simulink model "Bidirectional_AC_DC_full_control_V5_0_HW_Target"  (R2024a)
settings: Solver=VariableStepAuto  StartTime=0.0  StopTime=10.0  RelTol=1e-3
undefined symbols (not defined in the file): Down, GPTRIP1SEL, TZ1, Up
libraries: c2802xlib x7, c2837xDlib x7, simulink x5, slpidlib x3, spsFirstOrderFilterLib x2, spsAlphaBetaZerotodq0Lib x1
settings Model: Creator=MANSY  LastModifiedBy=MANSY

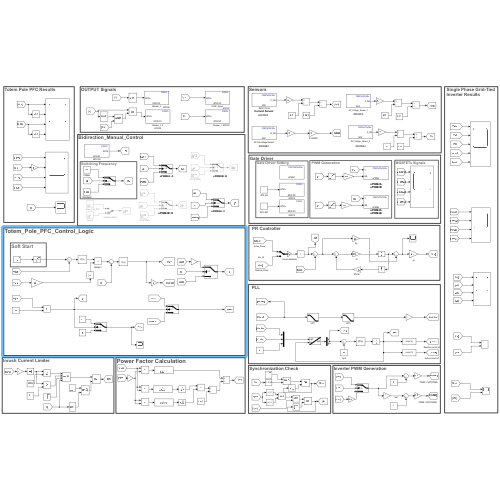
[thumbnail: Simulink's stored preview of the top-level diagram]
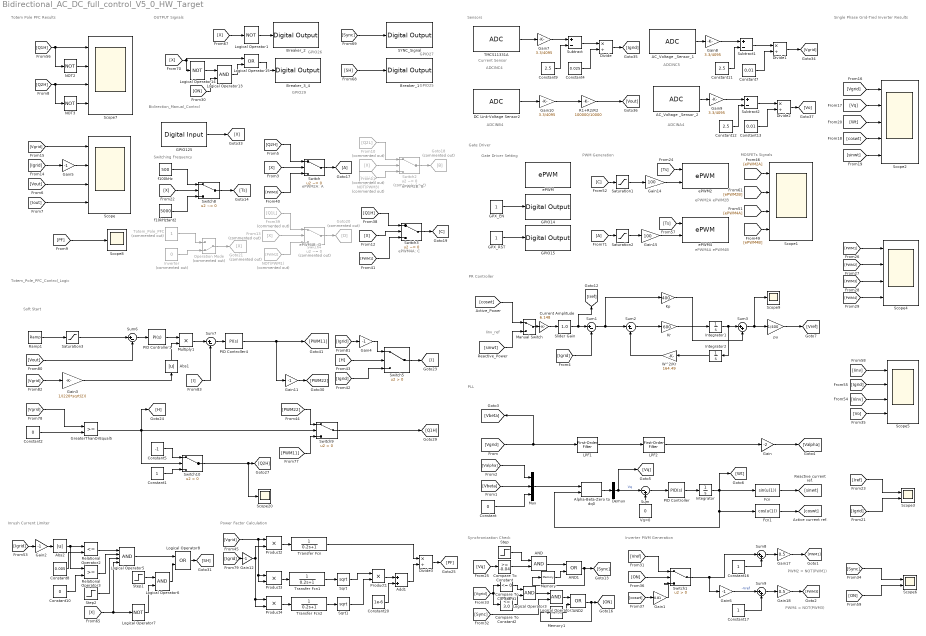
== system Bidirectional_AC_DC_full_control_V5_0_HW_Target ==
  note: Switching Frequency
  note: MOSFETs Signals
  note: OUTPUT Signals
  note: ePWM4A: C
  note: ePWM2B: B
  note: ePWM2A: A
  note: ADCINC5
  note: ADCINA4
  note: ADCINB4
  note: ADCINC4
  note: Synchronization Check
  note: PLL
  note: PR Controller
  note: Iinv_ref
  note: Bidirection_Manual_Control
  note: Inrush Current Limiter
  note: Sensors
  note: Current Sensor
  note: Gate Driver Setting
  note: ePWM2A
      | ePWM2B
  note: ePWM4A
      | ePWM4B
  note: PWM Generation
  note: Gate Driver
  note: ePWM4B: D
  note: GPIO29
  note: GPIO26
  note: GPIO27
  note: GPIO25
  note: Totem Pole PFC Results
  note: Single Phase Grid-Tied
      |  Inverter Results
  note: Soft Start
  note: Totem_Pole_PFC_Control_Logic
  note: Power Factor Calculation
  note: Inverter PWM Generation
  note: PWM2 = NOT(PWM1)
  note: PWM4 = NOT(PWM3)
  "          Totem_Pole_PFC" : Constant  Commented=on  OutDataTypeStr=boolean  SampleTime=1e-6
  AC_Voltage _Sensor_1 : c2802xlib/ADC  blkParamProc=C2000_Type4  ADCModule=C  samplingMode=Single sample mode  ADCResolution=12-bit (Single-ended input)  useSOC1=SOC1  useSOC2=SOC0_SOC1  SOCAcquisitionWindow=15  SOCTriggerSource=Software  SOCInterruptTrigger=No ADCINT  Ts=0.001  dType=uint16  postInterrupt=off  interruptSel=ADCINT1  ADCINTContinuous=on  endma=off  chdma=1  conv1=ADCINA0  conv2=ADCINA0 and ADCINB0  conv1_Type4=ADCIN5  conv2_Type4=ADCIN0 and ADCIN1
      settings: LibrarySourceBlock=c2837xDlib/ADC
  AC_Voltage _Sensor_2 : c2802xlib/ADC  blkParamProc=C2000_Type4  ADCModule=A  samplingMode=Single sample mode  ADCResolution=12-bit (Single-ended input)  useSOC1=SOC0  useSOC2=SOC0_SOC1  SOCAcquisitionWindow=15  SOCTriggerSource=Software  SOCInterruptTrigger=No ADCINT  Ts=0.001  dType=uint16  postInterrupt=off  interruptSel=ADCINT1  ADCINTContinuous=on  endma=off  chdma=1  conv1=ADCINA0  conv2=ADCINA0 and ADCINB0  conv1_Type4=ADCIN4  conv2_Type4=ADCIN0 and ADCIN1
      settings: LibrarySourceBlock=c2837xDlib/ADC
  AND : Logic  AllPortsSameDT=off  OutDataTypeStr=boolean
  AND1 : Logic  Operator=OR  AllPortsSameDT=off  OutDataTypeStr=boolean
  AND2 : Logic  Operator=OR  AllPortsSameDT=off  OutDataTypeStr=boolean
  Abs1 : Abs  SaturateOnIntegerOverflow=off
  Abs2 : Abs  SaturateOnIntegerOverflow=off
  Add1 : Sum
  Alpha-Beta-Zero to dq0 : spsAlphaBetaZerotodq0Lib/Alpha-Beta-Zero to dq0  Alignment=90 degrees behind phase A axis
  Breaker_1 : c2837xDlib/Digital Output  GPIO_Number=GPIO24~GPIO31  GPIO_Bit0=off  GPIO_BIT0_Toggle=off  GPIO_Bit1=on  GPIO_BIT1_Toggle=off  GPIO_Bit2=off  GPIO_BIT2_Toggle=off  GPIO_Bit3=off  GPIO_BIT3_Toggle=off  GPIO_Bit4=off  GPIO_BIT4_Toggle=off  GPIO_Bit5=off  GPIO_BIT5_Toggle=off  GPIO_Bit6=off  GPIO_BIT6_Toggle=off  GPIO_Bit7=off  GPIO_BIT7_Toggle=off
  Breaker_2 : c2837xDlib/Digital Output  GPIO_Number=GPIO24~GPIO31  GPIO_Bit0=off  GPIO_BIT0_Toggle=off  GPIO_Bit1=off  GPIO_BIT1_Toggle=off  GPIO_Bit2=on  GPIO_BIT2_Toggle=off  GPIO_Bit3=off  GPIO_BIT3_Toggle=off  GPIO_Bit4=off  GPIO_BIT4_Toggle=off  GPIO_Bit5=off  GPIO_BIT5_Toggle=off  GPIO_Bit6=off  GPIO_BIT6_Toggle=off  GPIO_Bit7=off  GPIO_BIT7_Toggle=off
  Breaker_3_4 : c2837xDlib/Digital Output  GPIO_Number=GPIO24~GPIO31  GPIO_Bit0=off  GPIO_BIT0_Toggle=off  GPIO_Bit1=off  GPIO_BIT1_Toggle=off  GPIO_Bit2=off  GPIO_BIT2_Toggle=off  GPIO_Bit3=off  GPIO_BIT3_Toggle=off  GPIO_Bit4=off  GPIO_BIT4_Toggle=off  GPIO_Bit5=on  GPIO_BIT5_Toggle=off  GPIO_Bit6=off  GPIO_BIT6_Toggle=off  GPIO_Bit7=off  GPIO_BIT7_Toggle=off
  Compare To Constant : simulink/Logic and Bit Operations/Compare To Constant  relop=>=  const=-0.04  OutDataTypeStr=boolean
  Compare To Constant1 : simulink/Logic and Bit Operations/Compare To Constant  relop=<=  const=0  OutDataTypeStr=boolean
  Compare To Constant2 : simulink/Logic and Bit Operations/Compare To Constant  relop=<=  const=3.0  OutDataTypeStr=boolean
  Constant : Constant  Value=0
  Constant1 : Constant
  Constant10 : Constant  Value=0
  Constant11 : Constant  Value=2.5
  Constant12 : Constant  Value=2.5
  Constant13 : Constant  Value=0.01
  Constant16 : Constant
  Constant17 : Constant
  Constant2 : Constant  Value=0
  Constant20 : Constant  Value=1e-6
  Constant4 : Constant  Value=0.025
  Constant5 : Constant  Value=-1
  Constant7 : Constant  Value=0.01
  Constant8 : Constant  Value=0.005
  Constant9 : Constant  Value=2.5
  Current Amplitude : Gain  Gain=6.148
  DC Link-Voltage Sensor2 : c2802xlib/ADC  blkParamProc=C2000_Type4  ADCModule=B  samplingMode=Single sample mode  ADCResolution=12-bit (Single-ended input)  useSOC1=SOC1  useSOC2=SOC0_SOC1  SOCAcquisitionWindow=15  SOCTriggerSource=Software  SOCInterruptTrigger=No ADCINT  Ts=0.001  dType=uint16  postInterrupt=off  interruptSel=ADCINT1  ADCINTContinuous=on  endma=off  chdma=1  conv1=ADCINA0  conv2=ADCINA0 and ADCINB0  conv1_Type4=ADCIN4  conv2_Type4=ADCIN0 and ADCIN1
      settings: LibrarySourceBlock=c2837xDlib/ADC
  Demux : Demux  Outputs=3
  Divide{,1..3} (4 alike) : Product  Inputs=*/
  Fcn : Fcn  Expr=sin(u(1))
  Fcn1 : Fcn  Expr=cos(u(1))
  From10 : From  Commented=on  GotoTag=Q2L
  From11 : From  Commented=on  GotoTag=X
  From13 : From  Commented=on  GotoTag=X
  From39 : From  Commented=on  GotoTag=Q1L
  From71 : From
  GPIO125 : c2837xDlib/Digital Input  GPIO_Number=GPIO120~GPIO127  GPIO_Bit0=off  GPIO_Bit1=off  GPIO_Bit2=off  GPIO_Bit3=off  GPIO_Bit4=off  GPIO_Bit5=on  GPIO_Bit6=off  GPIO_Bit7=off  sampleTime=0.1  dataType=auto  GPIO_Bit0_Qualification=Sync to SYSCLKOUT  GPIO_Bit1_Qualification=Sync to SYSCLKOUT  GPIO_Bit2_Qualification=Sync to SYSCLKOUT  GPIO_Bit3_Qualification=Sync to SYSCLKOUT  GPIO_Bit4_Qualification=Sync to SYSCLKOUT  GPIO_Bit5_Qualification=Sync to SYSCLKOUT  GPIO_Bit6_Qualification=Sync to SYSCLKOUT  GPIO_Bit7_Qualification=Sync to SYSCLKOUT  Qualification_Period=-1
  GPIO14 : c2837xDlib/Digital Output  GPIO_Number=GPIO8~GPIO15  GPIO_Bit0=off  GPIO_BIT0_Toggle=off  GPIO_Bit1=off  GPIO_BIT1_Toggle=off  GPIO_Bit2=off  GPIO_BIT2_Toggle=off  GPIO_Bit3=off  GPIO_BIT3_Toggle=off  GPIO_Bit4=off  GPIO_BIT4_Toggle=off  GPIO_Bit5=off  GPIO_BIT5_Toggle=off  GPIO_Bit6=on  GPIO_BIT6_Toggle=off  GPIO_Bit7=off  GPIO_BIT7_Toggle=off
  GPIO15 : c2837xDlib/Digital Output  GPIO_Number=GPIO8~GPIO15  GPIO_Bit0=off  GPIO_BIT0_Toggle=off  GPIO_Bit1=off  GPIO_BIT1_Toggle=off  GPIO_Bit2=off  GPIO_BIT2_Toggle=off  GPIO_Bit3=off  GPIO_BIT3_Toggle=off  GPIO_Bit4=off  GPIO_BIT4_Toggle=off  GPIO_Bit5=off  GPIO_BIT5_Toggle=off  GPIO_Bit6=off  GPIO_BIT6_Toggle=off  GPIO_Bit7=on  GPIO_BIT7_Toggle=off
  GPX_EN : Constant  SampleTime=1e-5
  GPX_RST : Constant  SampleTime=1e-5
  Gain : Gain  Gain=-2
  Gain1 : Gain  Gain=0.81
  Gain{7..10} (4 alike) : Gain  Gain=3.3/4095
  Gain{2,4..6,11..12} (6 alike) : Gain  Gain=-1
  Gain14 : Gain  Gain=100
  Gain15 : Gain  Gain=100
  Gain17 : Gain  Gain=0.5
  Gain18 : Gain  Gain=0.5
  Gain3 : Gain  Gain=1/(220*sqrt(2))
  Goto17 : Goto
  Goto18 : Goto  Commented=on  GotoTag=B
  Goto20 : Goto  Commented=on  GotoTag=D
  Goto21 : Goto  Commented=on  GotoTag=X
  GreaterThanOrEqual5 : RelationalOperator  OutDataTypeStr=boolean  RndMeth=Simplest  InputSameDT=off
  Integrator : Integrator
  Integrator1 : Integrator
  Integrator2 : Integrator
  Inverter : Constant  Commented=on  Value=0  OutDataTypeStr=boolean  SampleTime=1e-6
  Kp : Gain  Gain=400
  Kr : Gain  Gain=600
  LPF1 : spsFirstOrderFilterLib/First-Order Filter  FilterType=Lowpass  Tc=1/(2*pi*50)  Ts=0  Initialize=off  Vac_Init=[0, 0, 60]  Vdc_Init=0  PlotResponse=off  FreqRange="[0,  200,  1]"
  LPF2 : spsFirstOrderFilterLib/First-Order Filter  FilterType=Lowpass  Tc=1/(2*pi*50)  Ts=0  Initialize=off  Vac_Init=[0, 0, 60]  Vdc_Init=0  PlotResponse=off  FreqRange="[0,  200,  1]"
  Logical Operator1 : Logic  Operator=NOT  AllPortsSameDT=off  OutDataTypeStr=boolean
  Logical Operator{2..3,6,13} (4 alike) : Logic  AllPortsSameDT=off  OutDataTypeStr=boolean
  Logical Operator14 : Logic  Operator=NOT  AllPortsSameDT=off  OutDataTypeStr=boolean
  Logical Operator15 : Logic  Operator=OR  AllPortsSameDT=off  OutDataTypeStr=boolean
  Logical Operator5 : Logic  Inputs=4  AllPortsSameDT=off  OutDataTypeStr=boolean
  Logical Operator7 : Logic  Operator=NOT  AllPortsSameDT=off  OutDataTypeStr=boolean
  Logical Operator8 : Logic  Operator=OR  AllPortsSameDT=off  OutDataTypeStr=boolean
  Manual Switch : ManualSwitch
  Memory : Memory
  Memory1 : Memory
  Multiply1 : Product
  Mux : Mux  Inputs=3
  NOT(PWM1) : From  Commented=on  GotoTag=PWM2
  NOT(PWM3) : From  Commented=on  GotoTag=PWM4
  NOT2 : Logic  Operator=NOT  AllPortsSameDT=off  OutDataTypeStr=boolean
  NOT3 : Logic  Operator=NOT  AllPortsSameDT=off  OutDataTypeStr=boolean
  Operation Mode : ManualSwitch  Commented=on  CurrentSetting=0
  PID Controller : slpidlib/PID Controller  Controller=PID  Form=Parallel  TimeDomain=Continuous-time  UseExternalTs=off  SampleTime=-1  IntegratorMethod=Forward Euler  FilterMethod=Forward Euler  ControllerParametersSource=internal  P=100  I=10000  UseKiTs=off  D=0  UseExternalDerivativeSource=off  N=100  UseFilter=on  TunerSelectOption=Transfer Function Based (PID Tuner App)  InitialConditionSource=internal  InitialConditionForIntegrator=0  InitialConditionForFilter=0  DifferentiatorICPrevScaledInput=0  ExternalReset=none  TrackingMode=off  Kt=1  LimitOutput=off  SatLimitsSource=internal  UpperSaturationLimit=inf  LowerSaturationLimit=-inf  LinearizeAsGain=on  AntiWindupMode=none  Kb=1  LimitIntegrator=off  UpperIntegratorSaturationLimit=inf  LowerIntegratorSaturationLimit=-inf  POutMin=[]  POutMax=[]  IOutMin=[]  IOutMax=[]  DOutMin=[]  DOutMax=[]  NOutMin=[]  NOutMax=[]  SumOutMin=[]  SumOutMax=[]  SaturationOutMin=[]  SaturationOutMax=[]  PParamMin=[]  PParamMax=[]  IParamMin=[]  IParamMax=[]  DParamMin=[]  DParamMax=[]  NParamMin=[]  NParamMax=[]  KbParamMin=[]  KbParamMax=[]  KtParamMin=[]  KtParamMax=[]  KbOutMin=[]  KbOutMax=[]  KtOutMin=[]  KtOutMax=[]  IntegratorOutMin=[]  IntegratorOutMax=[]  FilterOutMin=[]  FilterOutMax=[]  SumI1OutMin=[]  SumI1OutMax=[]  SumI2OutMin=[]  SumI2OutMax=[]  SumI3OutMin=[]  SumI3OutMax=[]  SumI4OutMin=[]  SumI4OutMax=[]  SumDOutMin=[]  SumDOutMax=[]  DifferentiatorOutMin=[]  DifferentiatorOutMax=[]  FilterDiffOutCoefMin=[]  FilterDiffOutCoefMax=[]  ReciprocalOutMin=[]  ReciprocalOutMax=[]  SumDenOutMin=[]  SumDenOutMax=[]  SumNumOutMin=[]  SumNumOutMax=[]  DivideOutMin=[]  DivideOutMax=[]  UdiffTsProdOutMin=[]  UdiffTsProdOutMax=[]  NTsProdOutMin=[]  NTsProdOutMax=[]  UintegralTsProdOutMin=[]  UintegralTsProdOutMax=[]  UngainTsProdOutMin=[]  UngainTsProdOutMax=[]  ClampingZeroOutDataTypeStr=Inherit: Inherit via back propagation  ClampingZeroOutMin=[]  ClampingZeroOutMax=[]  FilterDenConstantOutDataTypeStr=Inherit: Inherit via back propagation  FilterDenConstantOutMin=[]  FilterDenConstantOutMax=[]  PCopyOutDataTypeStr=Inherit: Inherit via back propagation  PCopyOutMin=[]  PCopyOutMax=[]  NCopyOutDataTypeStr=Inherit: Inherit via back propagation  NCopyOutMin=[]  NCopyOutMax=[]  IntegratorContinuousStateAttributes=''  IntegratorStateMustResolveToSignalObject=off  IntegratorRTWStateStorageClass=Auto  FilterContinuousStateAttributes=''  FilterStateMustResolveToSignalObject=off  FilterRTWStateStorageClass=Auto  ParallelPVariant=InternalParameters  IdealPVariant=Disabled  IVariant=InternalParameters  DVariant=InternalParameters  IntegratorVariant=Continuous  SatVariant=Disabled  AWVariant=Passthrough  PCopyVariant=Disabled  TRVariant=Disabled  FdbkBlocksVariant=Forward  IdealPFdbkVariant=Disabled  SatFdbkVariant=Disabled  DerivativeFilterVariant=ContFilter  NVariant=InternalParameters  NCopyVariant=Disabled  FilterICVariant=InternalICsFilter  IntegratorICVariant=InternalICs  ExternalResetVariant=Disabled  TRSumVariant=Passthrough  SumFdbkVariant=Disabled  SumVariant=Sum_PID  TsampFilterVariant=InternalTs  TsampNgainVariant=Passthrough  TsampIntegralVariant=Disabled_SignalSpec  ExternalSaturationOutDataTypeStr=Inherit: Same as second input  DerivativeSourceVariant=ErrorSignal
  PID Controller1 : slpidlib/PID Controller  Controller=PI  Form=Parallel  TimeDomain=Continuous-time  UseExternalTs=off  SampleTime=-1  IntegratorMethod=Forward Euler  FilterMethod=Forward Euler  ControllerParametersSource=internal  P=.1  I=0.75  UseKiTs=off  D=0  UseExternalDerivativeSource=off  N=100  UseFilter=on  TunerSelectOption=Transfer Function Based (PID Tuner App)  InitialConditionSource=internal  InitialConditionForIntegrator=0  InitialConditionForFilter=0  DifferentiatorICPrevScaledInput=0  ExternalReset=none  TrackingMode=off  Kt=1  LimitOutput=off  SatLimitsSource=internal  UpperSaturationLimit=inf  LowerSaturationLimit=-inf  LinearizeAsGain=on  AntiWindupMode=none  Kb=1  LimitIntegrator=off  UpperIntegratorSaturationLimit=inf  LowerIntegratorSaturationLimit=-inf  POutMin=[]  POutMax=[]  IOutMin=[]  IOutMax=[]  DOutMin=[]  DOutMax=[]  NOutMin=[]  NOutMax=[]  SumOutMin=[]  SumOutMax=[]  SaturationOutMin=[]  SaturationOutMax=[]  PParamMin=[]  PParamMax=[]  IParamMin=[]  IParamMax=[]  DParamMin=[]  DParamMax=[]  NParamMin=[]  NParamMax=[]  KbParamMin=[]  KbParamMax=[]  KtParamMin=[]  KtParamMax=[]  KbOutMin=[]  KbOutMax=[]  KtOutMin=[]  KtOutMax=[]  IntegratorOutMin=[]  IntegratorOutMax=[]  FilterOutMin=[]  FilterOutMax=[]  SumI1OutMin=[]  SumI1OutMax=[]  SumI2OutMin=[]  SumI2OutMax=[]  SumI3OutMin=[]  SumI3OutMax=[]  SumI4OutMin=[]  SumI4OutMax=[]  SumDOutMin=[]  SumDOutMax=[]  DifferentiatorOutMin=[]  DifferentiatorOutMax=[]  FilterDiffOutCoefMin=[]  FilterDiffOutCoefMax=[]  ReciprocalOutMin=[]  ReciprocalOutMax=[]  SumDenOutMin=[]  SumDenOutMax=[]  SumNumOutMin=[]  SumNumOutMax=[]  DivideOutMin=[]  DivideOutMax=[]  UdiffTsProdOutMin=[]  UdiffTsProdOutMax=[]  NTsProdOutMin=[]  NTsProdOutMax=[]  UintegralTsProdOutMin=[]  UintegralTsProdOutMax=[]  UngainTsProdOutMin=[]  UngainTsProdOutMax=[]  ClampingZeroOutDataTypeStr=Inherit: Inherit via back propagation  ClampingZeroOutMin=[]  ClampingZeroOutMax=[]  FilterDenConstantOutDataTypeStr=Inherit: Inherit via back propagation  FilterDenConstantOutMin=[]  FilterDenConstantOutMax=[]  PCopyOutDataTypeStr=Inherit: Inherit via back propagation  PCopyOutMin=[]  PCopyOutMax=[]  NCopyOutDataTypeStr=Inherit: Inherit via back propagation  NCopyOutMin=[]  NCopyOutMax=[]  IntegratorContinuousStateAttributes=''  IntegratorStateMustResolveToSignalObject=off  IntegratorRTWStateStorageClass=Auto  FilterContinuousStateAttributes=''  FilterStateMustResolveToSignalObject=off  FilterRTWStateStorageClass=Auto  ParallelPVariant=InternalParameters  IdealPVariant=Disabled  IVariant=InternalParameters  DVariant=Disabled  IntegratorVariant=Continuous  SatVariant=Disabled  AWVariant=Passthrough  PCopyVariant=Disabled  TRVariant=Disabled  FdbkBlocksVariant=Forward  IdealPFdbkVariant=Disabled  SatFdbkVariant=Disabled  DerivativeFilterVariant=Disabled  NVariant=Disabled  NCopyVariant=Disabled_SignalSpec  FilterICVariant=Disabled  IntegratorICVariant=InternalICs  ExternalResetVariant=Disabled  TRSumVariant=Passthrough  SumFdbkVariant=Disabled  SumVariant=Sum_PI  TsampFilterVariant=InternalTs  TsampNgainVariant=Passthrough  TsampIntegralVariant=Disabled_SignalSpec  ExternalSaturationOutDataTypeStr=Inherit: Same as second input  DerivativeSourceVariant=Disabled
  PID Controller4 : slpidlib/PID Controller  Controller=PI  Form=Parallel  TimeDomain=Continuous-time  UseExternalTs=off  SampleTime=-1  IntegratorMethod=Forward Euler  FilterMethod=Forward Euler  ControllerParametersSource=internal  P=600  I=100  UseKiTs=off  D=0  UseExternalDerivativeSource=off  N=100  UseFilter=on  TunerSelectOption=Transfer Function Based (PID Tuner App)  InitialConditionSource=internal  InitialConditionForIntegrator=0  InitialConditionForFilter=0  DifferentiatorICPrevScaledInput=0  ExternalReset=none  TrackingMode=off  Kt=1  LimitOutput=off  SatLimitsSource=internal  UpperSaturationLimit=.99  LowerSaturationLimit=0  LinearizeAsGain=on  AntiWindupMode=none  Kb=1  LimitIntegrator=off  UpperIntegratorSaturationLimit=inf  LowerIntegratorSaturationLimit=-inf  POutMin=[]  POutMax=[]  IOutMin=[]  IOutMax=[]  DOutMin=[]  DOutMax=[]  NOutMin=[]  NOutMax=[]  SumOutMin=[]  SumOutMax=[]  SaturationOutMin=[]  SaturationOutMax=[]  PParamMin=[]  PParamMax=[]  IParamMin=[]  IParamMax=[]  DParamMin=[]  DParamMax=[]  NParamMin=[]  NParamMax=[]  KbParamMin=[]  KbParamMax=[]  KtParamMin=[]  KtParamMax=[]  KbOutMin=[]  KbOutMax=[]  KtOutMin=[]  KtOutMax=[]  IntegratorOutMin=[]  IntegratorOutMax=[]  FilterOutMin=[]  FilterOutMax=[]  SumI1OutMin=[]  SumI1OutMax=[]  SumI2OutMin=[]  SumI2OutMax=[]  SumI3OutMin=[]  SumI3OutMax=[]  SumI4OutMin=[]  SumI4OutMax=[]  SumDOutMin=[]  SumDOutMax=[]  DifferentiatorOutMin=[]  DifferentiatorOutMax=[]  FilterDiffOutCoefMin=[]  FilterDiffOutCoefMax=[]  ReciprocalOutMin=[]  ReciprocalOutMax=[]  SumDenOutMin=[]  SumDenOutMax=[]  SumNumOutMin=[]  SumNumOutMax=[]  DivideOutMin=[]  DivideOutMax=[]  UdiffTsProdOutMin=[]  UdiffTsProdOutMax=[]  NTsProdOutMin=[]  NTsProdOutMax=[]  UintegralTsProdOutMin=[]  UintegralTsProdOutMax=[]  UngainTsProdOutMin=[]  UngainTsProdOutMax=[]  ClampingZeroOutDataTypeStr=Inherit: Inherit via back propagation  ClampingZeroOutMin=[]  ClampingZeroOutMax=[]  FilterDenConstantOutDataTypeStr=Inherit: Inherit via back propagation  FilterDenConstantOutMin=[]  FilterDenConstantOutMax=[]  PCopyOutDataTypeStr=Inherit: Inherit via back propagation  PCopyOutMin=[]  PCopyOutMax=[]  NCopyOutDataTypeStr=Inherit: Inherit via back propagation  NCopyOutMin=[]  NCopyOutMax=[]  IntegratorContinuousStateAttributes=''  IntegratorStateMustResolveToSignalObject=off  IntegratorRTWStateStorageClass=Auto  FilterContinuousStateAttributes=''  FilterStateMustResolveToSignalObject=off  FilterRTWStateStorageClass=Auto  ParallelPVariant=InternalParameters  IdealPVariant=Disabled  IVariant=InternalParameters  DVariant=Disabled  IntegratorVariant=Continuous  SatVariant=Disabled  AWVariant=Passthrough  PCopyVariant=Disabled  TRVariant=Disabled  FdbkBlocksVariant=Forward  IdealPFdbkVariant=Disabled  SatFdbkVariant=Disabled  DerivativeFilterVariant=Disabled  NVariant=Disabled  NCopyVariant=Disabled_SignalSpec  FilterICVariant=Disabled  IntegratorICVariant=InternalICs  ExternalResetVariant=Disabled  TRSumVariant=Passthrough  SumFdbkVariant=Disabled  SumVariant=Sum_PI  TsampFilterVariant=InternalTs  TsampNgainVariant=Passthrough  TsampIntegralVariant=Disabled_SignalSpec  ExternalSaturationOutDataTypeStr=Inherit: Same as second input  DerivativeSourceVariant=Disabled
  Product{1..4} (4 alike) : Product
  R1+R2/R2 : Gain  Gain=100000/10000
  Ramp1 : simulink/Sources/Ramp  slope=4000  start=0  InitialOutput=0
  Relational Operator2 : RelationalOperator  Operator=<=  OutDataTypeStr=boolean  RndMeth=Simplest  InputSameDT=off
  Relational Operator3 : RelationalOperator  OutDataTypeStr=boolean  RndMeth=Simplest  InputSameDT=off
  "SYNC_Signal  " : c2837xDlib/Digital Output  GPIO_Number=GPIO24~GPIO31  GPIO_Bit0=off  GPIO_BIT0_Toggle=off  GPIO_Bit1=off  GPIO_BIT1_Toggle=off  GPIO_Bit2=off  GPIO_BIT2_Toggle=off  GPIO_Bit3=on  GPIO_BIT3_Toggle=off  GPIO_Bit4=off  GPIO_BIT4_Toggle=off  GPIO_Bit5=off  GPIO_BIT5_Toggle=off  GPIO_Bit6=off  GPIO_BIT6_Toggle=off  GPIO_Bit7=off  GPIO_BIT7_Toggle=off
  Saturation1 : Saturate  UpperLimit=1  LowerLimit=0
  Saturation2 : Saturate  UpperLimit=1  LowerLimit=0
  Saturation3 : Saturate  UpperLimit=400  LowerLimit=0
  Scope{,1,4..5,7} (5 alike) : Scope  NumInputPorts=4
  Scope2 : Scope  NumInputPorts=5
  Scope20 : Scope
  Scope3 : Scope  NumInputPorts=2
  Scope6 : Scope  NumInputPorts=2
  Scope8 : Scope
  Scope9 : Scope
  Slider Gain : simulink/Math Operations/Slider Gain  gain=1.0  low=0  high=1
  Sqrt : Sqrt
  Sqrt1 : Sqrt
  Step : Step  Time=0.02  SampleTime=0
  Step1 : Step  Time=0.005  SampleTime=0
  Step2 : Step  Time=0.14  SampleTime=0
  Subtract : Sum  Inputs=+-
  Subtract1 : Sum  Inputs=+-
  Subtract2 : Sum  Inputs=+-
  Sum : Sum  Inputs=|-+
  Sum{1..2,6..7} (4 alike) : Sum  Inputs=|+-
  Sum3 : Sum  Inputs=|++
  Sum8 : Sum  Inputs=|++
  Sum9 : Sum  Inputs=|++
  Switch : Switch  Criteria=u2 ~= 0  SaturateOnIntegerOverflow=off  InputSameDT=off
  Switch{1,5,9..10} (4 alike) : Switch  Criteria=u2 > Threshold  SaturateOnIntegerOverflow=off  InputSameDT=off
  Switch2 : Switch  Commented=on  Criteria=u2 ~= 0  SaturateOnIntegerOverflow=off  InputSameDT=off
  Switch3 : Switch  Criteria=u2 ~= 0  SaturateOnIntegerOverflow=off  InputSameDT=off
  Switch4 : Switch  Commented=on  Criteria=u2 ~= 0  SaturateOnIntegerOverflow=off  InputSameDT=off
  Switch8 : Switch  Criteria=u2 ~= 0  SaturateOnIntegerOverflow=off  InputSameDT=off
  TMCS11331A : c2802xlib/ADC  blkParamProc=C2000_Type4  ADCModule=C  samplingMode=Single sample mode  ADCResolution=12-bit (Single-ended input)  useSOC1=SOC0  useSOC2=SOC0_SOC1  SOCAcquisitionWindow=15  SOCTriggerSource=Software  SOCInterruptTrigger=No ADCINT  Ts=0.001  dType=uint16  postInterrupt=off  interruptSel=ADCINT1  ADCINTContinuous=on  endma=off  chdma=1  conv1=ADCINA0  conv2=ADCINA0 and ADCINB0  conv1_Type4=ADCIN4  conv2_Type4=ADCIN0 and ADCIN1
      settings: LibrarySourceBlock=c2837xDlib/ADC
  Transfer Fcn : TransferFcn  Denominator=[0.2 1]
  Transfer Fcn1 : TransferFcn  Denominator=[0.2 1]
  Transfer Fcn2 : TransferFcn  Denominator=[0.2 1]
  Vq=0 : Constant  Value=0
  W^2/Kr : Gain  Gain=164.49
  ePWM : c2802xlib/ePWM  PwmType=C2000_Type4  useModule=ePWM1  ePWMxLINKTBPRD=Not Linked  periodUnits=Clock cycles  timerSource=Specify via dialog  timerPeriod_clk=100  timerPeriod_sec=0.0001  tbshadow=Counter equals to zero  countingMode=Up-Down  phaseActiveEnable=Disable  phaseDirection=Count down after sync  phaseActive=0  synchronizationEnable=off  dcaevt1Sync=off  dcbevt1Sync=off  synchronizationOption=Disable  dcbevt1SyncOut=off  dcaevt1SyncOut=off  cmpdSyncOut=off  cmpcSyncOut=off  cmpbSyncOut=off  zeroSyncOut=off  swfSyncOut=off  perSynchronizationOption=Counter equals to period (CTR=PRD)  clockPrescale=1  HSclockPrescale=1  enswap=off  ePWMxAStatus=on  ePWMxAactionLogic1=Do nothing  ePWMxAactionLogic2=Do nothing  ePWMxAactionLogic3=Clear  ePWMxAactionLogic4=Set  ePWMxAactionLogic5=Do nothing  ePWMxAactionLogic6=Do nothing  ePWMxACSFenable=off  ePWMxACSFvalue=Forcing disable  ePWMxASFreload=Zero  ePWMxBStatus=on  ePWMxBactionLogic1=Do nothing  ePWMxBactionLogic2=Do nothing  ePWMxBactionLogic3=Set  ePWMxBactionLogic4=Clear  ePWMxBactionLogic5=Do nothing  ePWMxBactionLogic6=Do nothing  ePWMxBCSFenable=off  ePWMxBCSFvalue=Forcing disable  ePWMxBSFreload=Zero  ePWNxBOutWay=off  ePWMxLINKCMPA=Not Linked  CMPAUnits=Percentages  CMPASource=Specify via dialog  CMPAValue_per=50  CMPAValue_clk=32000  enCMPAshadow=Counter equals to zero (CTR=Zero)  ePWMxLINKCMPB=Not Linked  CMPBUnits=Percentages  CMPBSource=Specify via dialog  CMPBValue_per=50  CMPBValue_clk=50  enCMPBshadow=Counter equals to zero (CTR=Zero)  ePWMxLINKCMPC=Not Linked  CMPCUnits=Clock cycles  CMPCSource=Specify via dialog  CMPCValue_per=50  CMPCValue_clk=32000  enCMPCshadow=Counter equals to zero (CTR=Zero)  ePWMxLINKCMPD=Not Linked  CMPDUnits=Clock cycles  CMPDSource=Specify via dialog  CMPDValue_per=50  CMPDValue_clk=32000  enCMPDshadow=Counter equals to zero (CTR=Zero)  enableDBePWMxA=on  enableDBePWMxB=on  enhalfcycle=off  DBpolarity=Active high complementary (AHC)  DBedgeDelay=Positive  DBSource_ePWMxA=ePWMxA  DBSource_ePWMxB=ePWMxA  DBPeriodUnits=Clock cycles  DBperiodSource=Specify via dialog  REDperiod=5  FEDperiod=5  REDperiod_sec=0  FEDperiod_sec=0  LoadModeDBRED=Immediate without using shadow  LoadModeDBFED=Immediate without using shadow  adcstartModuleA=off  adcrequestEventA=First event  adcstartEventA=Digital Compare Module A Event 1 start of conversion (DCAEVT1.soc)  adcstartEventA_type2=Counter equals to zero (CTR=Zero)  adcstartModuleB=off  adcrequestEventB=First event  adcstartEventB=Counter equals to zero (CTR=Zero)  adcstartEventB_type2=Counter equals to zero (CTR=Zero)  intEn=off  intPrd=First event  intSel=Counter equals to zero (CTR=Zero)  intSel_type2=Counter equals to zero (CTR=Zero)  hrpe=off  enHRPWM=off  HRPWM_LoadMode=Counter equals to period (CTR=PRD)  HRPWM_CTLMode=Duty or Period control mode  HRPWM_EDGMode=Both edge  hrpeb=off  enHRPWMB=off  HRPWM_LoadModeB=Counter equals to zero (CTR=ZERO)  HRPWM_CTLModeB=Duty or Period control mode  HRPWM_EDGModeB=Both edge  enHRDBRED=off  enHRDBFED=off  enSFO=on  enautoconv=on  chopperEnable=off  chopperFrequency=1  chopperFirstwidth=1  chopperDuty=12.5%  tripZonesource=Specify via dialog  tzselOSHT1=off  tzselOSHT2=off  tzselOSHT3=off  tzselOSHT4=off  tzselOSHT5=off  tzselOSHT6=off  tzselOSHDCAEV1=off  tzselOSHDCBEV1=off  tzselCBC1=off  tzselCBC2=off  tzselCBC3=off  tzselCBC4=off  tzselCBC5=off  tzselCBC6=off  tzselCBCDCAEV2=off  tzselCBCDCBEV2=off  enTzOstIntr=off  enTzCbcIntr=off  enTzDCAEVT1Intr=off  enTzDCAEVT2Intr=off  enTzDCBEVT1Intr=off  enTzDCBEVT2Intr=off  tzclrCBCLatch=Counter equals to zero (CTR=Zero)  ePWMxAforced=No action  ePWMxBforced=No action  DCAEVT1forced=No action  DCBEVT1forced=No action  DCAEVT2forced=No action  DCBEVT2forced=No action  dcah=Trip Zone 1 input (TZ1)  dcal=Trip Zone 2 input (TZ2)  dcbh=Trip Zone 1 input (TZ1)  dcbl=Trip Zone 2 input (TZ2)  dcah_type2=GPTRIP1SEL/(TZ1)  dcal_type2=GPTRIP1SEL/(TZ1)  dcbh_type2=GPTRIP1SEL/(TZ1)  dcbl_type2=GPTRIP1SEL/(TZ1)  gendcaevt1=Event disabled  gendcaevt2=Event disabled  gendcbevt1=Event disabled  gendcbevt2=Event disabled  dcaevt1src=DCAEVT1 with sync  dcaevt2src=DCAEVT2 with sync  dcbevt1src=DCBEVT1 with sync  dcbevt2src=DCBEVT2 with sync  pulsesel=Counter equals to zero (CTR=Zero)  blankinv=off  blankoffset=0  blankwidth=0  evsrcsel=Filtered version of DCAEVT1 (DCAEVT1FILT)  encape=off
      settings: LibrarySourceBlock=c2837xDlib/ePWM
  ePWM2 : c2802xlib/ePWM  PwmType=C2000_Type4  useModule=ePWM2  ePWMxLINKTBPRD=Not Linked  periodUnits=Clock cycles  timerSource=Input port  timerPeriod_clk=0  timerPeriod_sec=0.0001  tbshadow=Counter equals to zero  countingMode=Up-Down  phaseActiveEnable=Disable  phaseDirection=Count down after sync  phaseActive=0  synchronizationEnable=off  dcaevt1Sync=off  dcbevt1Sync=off  synchronizationOption=Disable  dcbevt1SyncOut=off  dcaevt1SyncOut=off  cmpdSyncOut=off  cmpcSyncOut=off  cmpbSyncOut=off  zeroSyncOut=off  swfSyncOut=off  perSynchronizationOption=Counter equals to period (CTR=PRD)  clockPrescale=1  HSclockPrescale=1  enswap=off  ePWMxAStatus=on  ePWMxAactionLogic1=Do nothing  ePWMxAactionLogic2=Do nothing  ePWMxAactionLogic3=Clear  ePWMxAactionLogic4=Set  ePWMxAactionLogic5=Do nothing  ePWMxAactionLogic6=Do nothing  ePWMxACSFenable=off  ePWMxACSFvalue=Forcing disable  ePWMxASFreload=Zero  ePWMxBStatus=on  ePWMxBactionLogic1=Do nothing  ePWMxBactionLogic2=Do nothing  ePWMxBactionLogic3=Set  ePWMxBactionLogic4=Clear  ePWMxBactionLogic5=Do nothing  ePWMxBactionLogic6=Do nothing  ePWMxBCSFenable=off  ePWMxBCSFvalue=Forcing disable  ePWMxBSFreload=Zero  ePWNxBOutWay=on  ePWMxLINKCMPA=Not Linked  CMPAUnits=Percentages  CMPASource=Input port  CMPAValue_per=0  CMPAValue_clk=32000  enCMPAshadow=Counter equals to zero (CTR=Zero)  ePWMxLINKCMPB=Not Linked  CMPBUnits=Percentages  CMPBSource=Specify via dialog  CMPBValue_per=50  CMPBValue_clk=32000  enCMPBshadow=Counter equals to zero (CTR=Zero)  ePWMxLINKCMPC=Not Linked  CMPCUnits=Clock cycles  CMPCSource=Specify via dialog  CMPCValue_per=50  CMPCValue_clk=32000  enCMPCshadow=Counter equals to zero (CTR=Zero)  ePWMxLINKCMPD=Not Linked  CMPDUnits=Clock cycles  CMPDSource=Specify via dialog  CMPDValue_per=50  CMPDValue_clk=32000  enCMPDshadow=Counter equals to zero (CTR=Zero)  enableDBePWMxA=on  enableDBePWMxB=on  enhalfcycle=off  DBpolarity=Active high complementary (AHC)  DBedgeDelay=Positive  DBSource_ePWMxA=ePWMxA  DBSource_ePWMxB=ePWMxA  DBPeriodUnits=Clock cycles  DBperiodSource=Specify via dialog  REDperiod=100  FEDperiod=100  REDperiod_sec=0  FEDperiod_sec=0  LoadModeDBRED=Immediate without using shadow  LoadModeDBFED=Immediate without using shadow  adcstartModuleA=off  adcrequestEventA=First event  adcstartEventA=Digital Compare Module A Event 1 start of conversion (DCAEVT1.soc)  adcstartEventA_type2=Counter equals to zero (CTR=Zero)  adcstartModuleB=off  adcrequestEventB=First event  adcstartEventB=Counter equals to zero (CTR=Zero)  adcstartEventB_type2=Counter equals to zero (CTR=Zero)  intEn=off  intPrd=First event  intSel=Counter equals to zero (CTR=Zero)  intSel_type2=Counter equals to zero (CTR=Zero)  hrpe=off  enHRPWM=off  HRPWM_LoadMode=Counter equals to period (CTR=PRD)  HRPWM_CTLMode=Duty or Period control mode  HRPWM_EDGMode=Both edge  hrpeb=off  enHRPWMB=off  HRPWM_LoadModeB=Counter equals to zero (CTR=ZERO)  HRPWM_CTLModeB=Duty or Period control mode  HRPWM_EDGModeB=Both edge  enHRDBRED=off  enHRDBFED=off  enSFO=on  enautoconv=on  chopperEnable=off  chopperFrequency=1  chopperFirstwidth=1  chopperDuty=12.5%  tripZonesource=Specify via dialog  tzselOSHT1=off  tzselOSHT2=off  tzselOSHT3=off  tzselOSHT4=off  tzselOSHT5=off  tzselOSHT6=off  tzselOSHDCAEV1=off  tzselOSHDCBEV1=off  tzselCBC1=off  tzselCBC2=off  tzselCBC3=off  tzselCBC4=off  tzselCBC5=off  tzselCBC6=off  tzselCBCDCAEV2=off  tzselCBCDCBEV2=off  enTzOstIntr=off  enTzCbcIntr=off  enTzDCAEVT1Intr=off  enTzDCAEVT2Intr=off  enTzDCBEVT1Intr=off  enTzDCBEVT2Intr=off  tzclrCBCLatch=Counter equals to zero (CTR=Zero)  ePWMxAforced=No action  ePWMxBforced=No action  DCAEVT1forced=No action  DCBEVT1forced=No action  DCAEVT2forced=No action  DCBEVT2forced=No action  dcah=Trip Zone 1 input (TZ1)  dcal=Trip Zone 2 input (TZ2)  dcbh=Trip Zone 1 input (TZ1)  dcbl=Trip Zone 2 input (TZ2)  dcah_type2=GPTRIP1SEL/(TZ1)  dcal_type2=GPTRIP1SEL/(TZ1)  dcbh_type2=GPTRIP1SEL/(TZ1)  dcbl_type2=GPTRIP1SEL/(TZ1)  gendcaevt1=Event disabled  gendcaevt2=Event disabled  gendcbevt1=Event disabled  gendcbevt2=Event disabled  dcaevt1src=DCAEVT1 with sync  dcaevt2src=DCAEVT2 with sync  dcbevt1src=DCBEVT1 with sync  dcbevt2src=DCBEVT2 with sync  pulsesel=Counter equals to zero (CTR=Zero)  blankinv=off  blankoffset=0  blankwidth=0  evsrcsel=Filtered version of DCAEVT1 (DCAEVT1FILT)  encape=off
      settings: LibrarySourceBlock=c2837xDlib/ePWM
  ePWM4 : c2802xlib/ePWM  PwmType=C2000_Type4  useModule=ePWM4  ePWMxLINKTBPRD=Not Linked  periodUnits=Clock cycles  timerSource=Input port  timerPeriod_clk=0  timerPeriod_sec=0.0001  tbshadow=Counter equals to zero  countingMode=Up-Down  phaseActiveEnable=Disable  phaseDirection=Count down after sync  phaseActive=0  synchronizationEnable=off  dcaevt1Sync=off  dcbevt1Sync=off  synchronizationOption=Disable  dcbevt1SyncOut=off  dcaevt1SyncOut=off  cmpdSyncOut=off  cmpcSyncOut=off  cmpbSyncOut=off  zeroSyncOut=off  swfSyncOut=off  perSynchronizationOption=Counter equals to period (CTR=PRD)  clockPrescale=1  HSclockPrescale=1  enswap=off  ePWMxAStatus=on  ePWMxAactionLogic1=Do nothing  ePWMxAactionLogic2=Do nothing  ePWMxAactionLogic3=Clear  ePWMxAactionLogic4=Set  ePWMxAactionLogic5=Do nothing  ePWMxAactionLogic6=Do nothing  ePWMxACSFenable=off  ePWMxACSFvalue=Forcing disable  ePWMxASFreload=Zero  ePWMxBStatus=on  ePWMxBactionLogic1=Do nothing  ePWMxBactionLogic2=Do nothing  ePWMxBactionLogic3=Set  ePWMxBactionLogic4=Clear  ePWMxBactionLogic5=Do nothing  ePWMxBactionLogic6=Do nothing  ePWMxBCSFenable=off  ePWMxBCSFvalue=Forcing disable  ePWMxBSFreload=Zero  ePWNxBOutWay=on  ePWMxLINKCMPA=Not Linked  CMPAUnits=Percentages  CMPASource=Input port  CMPAValue_per=0  CMPAValue_clk=32000  enCMPAshadow=Counter equals to zero (CTR=Zero)  ePWMxLINKCMPB=Not Linked  CMPBUnits=Percentages  CMPBSource=Specify via dialog  CMPBValue_per=50  CMPBValue_clk=32000  enCMPBshadow=Counter equals to zero (CTR=Zero)  ePWMxLINKCMPC=Not Linked  CMPCUnits=Clock cycles  CMPCSource=Specify via dialog  CMPCValue_per=50  CMPCValue_clk=32000  enCMPCshadow=Counter equals to zero (CTR=Zero)  ePWMxLINKCMPD=Not Linked  CMPDUnits=Clock cycles  CMPDSource=Specify via dialog  CMPDValue_per=50  CMPDValue_clk=32000  enCMPDshadow=Counter equals to zero (CTR=Zero)  enableDBePWMxA=on  enableDBePWMxB=on  enhalfcycle=off  DBpolarity=Active high complementary (AHC)  DBedgeDelay=Positive  DBSource_ePWMxA=ePWMxA  DBSource_ePWMxB=ePWMxA  DBPeriodUnits=Clock cycles  DBperiodSource=Specify via dialog  REDperiod=100  FEDperiod=100  REDperiod_sec=0  FEDperiod_sec=0  LoadModeDBRED=Immediate without using shadow  LoadModeDBFED=Immediate without using shadow  adcstartModuleA=off  adcrequestEventA=First event  adcstartEventA=Digital Compare Module A Event 1 start of conversion (DCAEVT1.soc)  adcstartEventA_type2=Counter equals to zero (CTR=Zero)  adcstartModuleB=off  adcrequestEventB=First event  adcstartEventB=Counter equals to zero (CTR=Zero)  adcstartEventB_type2=Counter equals to zero (CTR=Zero)  intEn=off  intPrd=First event  intSel=Counter equals to zero (CTR=Zero)  intSel_type2=Counter equals to zero (CTR=Zero)  hrpe=off  enHRPWM=off  HRPWM_LoadMode=Counter equals to period (CTR=PRD)  HRPWM_CTLMode=Duty or Period control mode  HRPWM_EDGMode=Both edge  hrpeb=off  enHRPWMB=off  HRPWM_LoadModeB=Counter equals to zero (CTR=ZERO)  HRPWM_CTLModeB=Duty or Period control mode  HRPWM_EDGModeB=Both edge  enHRDBRED=off  enHRDBFED=off  enSFO=on  enautoconv=on  chopperEnable=off  chopperFrequency=1  chopperFirstwidth=1  chopperDuty=12.5%  tripZonesource=Specify via dialog  tzselOSHT1=off  tzselOSHT2=off  tzselOSHT3=off  tzselOSHT4=off  tzselOSHT5=off  tzselOSHT6=off  tzselOSHDCAEV1=off  tzselOSHDCBEV1=off  tzselCBC1=off  tzselCBC2=off  tzselCBC3=off  tzselCBC4=off  tzselCBC5=off  tzselCBC6=off  tzselCBCDCAEV2=off  tzselCBCDCBEV2=off  enTzOstIntr=off  enTzCbcIntr=off  enTzDCAEVT1Intr=off  enTzDCAEVT2Intr=off  enTzDCBEVT1Intr=off  enTzDCBEVT2Intr=off  tzclrCBCLatch=Counter equals to zero (CTR=Zero)  ePWMxAforced=No action  ePWMxBforced=No action  DCAEVT1forced=No action  DCBEVT1forced=No action  DCAEVT2forced=No action  DCBEVT2forced=No action  dcah=Trip Zone 1 input (TZ1)  dcal=Trip Zone 2 input (TZ2)  dcbh=Trip Zone 1 input (TZ1)  dcbl=Trip Zone 2 input (TZ2)  dcah_type2=GPTRIP1SEL/(TZ1)  dcal_type2=GPTRIP1SEL/(TZ1)  dcbh_type2=GPTRIP1SEL/(TZ1)  dcbl_type2=GPTRIP1SEL/(TZ1)  gendcaevt1=Event disabled  gendcaevt2=Event disabled  gendcbevt1=Event disabled  gendcbevt2=Event disabled  dcaevt1src=DCAEVT1 with sync  dcaevt2src=DCAEVT2 with sync  dcbevt1src=DCBEVT1 with sync  dcbevt2src=DCBEVT2 with sync  pulsesel=Counter equals to zero (CTR=Zero)  blankinv=off  blankoffset=0  blankwidth=0  evsrcsel=Filtered version of DCAEVT1 (DCAEVT1FILT)  encape=off
      settings: LibrarySourceBlock=c2837xDlib/ePWM
  f100kHz : Constant  Value=500
  f10kHztant2 : Constant  Value=5000
  pu : Gain  Gain=1/400
  wires:
  [X] -> Logical Operator5/4, Logical Operator7/1
  Logical Operator8/1 -> [SH]
  Step1/1 -> Logical Operator6/1
  Memory1/1 -> AND2/2
  [Igrid] -> Gain2/1
  Abs2/1 -> Relational Operator3/1, Relational Operator2/1
  Relational Operator2/1 -> Logical Operator5/1
  Logical Operator5/1 -> Logical Operator8/1
  Demux/2 -> Sum/1, [Vq]  "Vq"
  Mux/1 -> Alpha-Beta-Zero to dq0/1
  Fcn1/1 -> [coswt]
  From11/1 -> Switch2/2
  Gain2/1 -> Abs2/1
  Logical Operator6/1 -> Logical Operator8/2
  NOT(PWM1)/1 -> Switch4/3
  Switch4/1 -> Goto20/1
  [PWM1] -> Switch3/3
  [Q1H] -> Switch3/1
  Integrator1/1 -> Integrator2/1, Sum3/1
  "          Totem_Pole_PFC"/1 -> Operation Mode/1
  Slider Gain/1 -> [Iref], Sum1/1
  pu/1 -> [Vref]
  Constant8/1 -> Relational Operator2/2
  AND/1 -> AND1/1
  [X] -> Switch/2
  From10/1 -> Switch2/1
  Switch2/1 -> Goto18/1
  [sinwt] -> Manual Switch/2
  [X] -> Switch3/2
  NOT(PWM3)/1 -> Switch2/3
  W^2/Kr/1 -> Sum2/2
  Relational Operator3/1 -> Logical Operator5/2
  AND1/1 -> [Sync], Memory/1
  Logical Operator2/1 -> AND2/1
  From13/1 -> Switch4/2
  Operation Mode/1 -> Goto21/1
  Step/1 -> AND/1
  [Q2H] -> Switch/1
  Inverter/1 -> Operation Mode/2
  From39/1 -> Switch4/1
  Switch/1 -> Goto17/1
  Switch3/1 -> [C]
  Sum1/1 -> Sum2/1, Kp/1
  Fcn/1 -> [sinwt]
  Compare To Constant/1 -> AND/2
  Compare To Constant1/1 -> Logical Operator3/1
  Constant10/1 -> Relational Operator3/2
  [Vq] -> Compare To Constant/1
  AND2/1 -> Memory1/1, [ON]
  PID Controller/1 -> Integrator/1
  Memory/1 -> AND1/2
  Current Amplitude/1 -> Slider Gain/1
  LPF2/1 -> Gain/1
  Kr/1 -> Integrator1/1
  [PWM3] -> Switch/3
  Integrator/1 -> [Wt], Fcn/1, Fcn1/1, Alpha-Beta-Zero to dq0/2
  Manual Switch/1 -> Current Amplitude/1
  Alpha-Beta-Zero to dq0/1 -> Demux/1
  LPF1/1 -> LPF2/1
  [Valpha] -> Mux/1
  [coswt] -> Manual Switch/1
  Sum/1 -> PID Controller/1
  Step2/1 -> Logical Operator5/3
  Vq=0/1 -> Sum/2
  Logical Operator7/1 -> Logical Operator6/2
  Integrator2/1 -> W^2/Kr/1
  Sum2/1 -> Kr/1
  Sum3/1 -> Scope9/1, pu/1
  [Vbeta] -> Mux/2
  Compare To Constant2/1 -> Logical Operator3/2
  Constant/1 -> Mux/3
  [Vgrid] -> Compare To Constant2/1, Compare To Constant1/1
  [Igrid] -> Sum1/2
  Gain/1 -> [Valpha]
  [Vgrid] -> [Vbeta], LPF1/1
  Kp/1 -> Sum3/2
  Subtract/1 -> Divide/1
  Constant9/1 -> Subtract/2
  Gain7/1 -> Subtract/1
  TMCS11331A/1 -> Gain7/1
  Constant4/1 -> Divide/2
  Divide/1 -> [Igrid]
  AC_Voltage _Sensor_1/1 -> Gain8/1
  Constant11/1 -> Subtract1/2
  Constant7/1 -> Divide1/2
  Subtract1/1 -> Divide1/1
  Gain8/1 -> Subtract1/1
  Divide1/1 -> [Vgrid]
  Divide2/1 -> [Vo]
  Gain9/1 -> Subtract2/1
  Subtract2/1 -> Divide2/1
  Constant13/1 -> Divide2/2
  Constant12/1 -> Subtract2/2
  AC_Voltage _Sensor_2/1 -> Gain9/1
  DC Link-Voltage Sensor2/1 -> Gain10/1
  R1+R2/R2/1 -> [Vout]
  Gain10/1 -> R1+R2/R2/1
  GPIO125/1 -> [X]
  [C] -> Saturation1/1
  GPX_EN/1 -> GPIO14/1
  GPX_RST/1 -> GPIO15/1
  From71/1 -> Saturation2/1
  Saturation1/1 -> Gain14/1
  Saturation2/1 -> Gain15/1
  Logical Operator15/1 -> Breaker_3_4/1
  Logical Operator1/1 -> Breaker_2/1
  [X] -> Logical Operator15/1, Logical Operator14/1
  Logical Operator14/1 -> Logical Operator13/1
  [ON] -> Logical Operator13/2
  Logical Operator13/1 -> Logical Operator15/2
  [SH] -> Breaker_1/1
  [X] -> Logical Operator1/1
  [Sync] -> "SYNC_Signal  "/1
  Gain15/1 -> ePWM4/2
  Gain14/1 -> ePWM2/2
  [Ts] -> ePWM2/1
  [Ts] -> ePWM4/1
  [Iout] -> Scope/4
  [Vgrid] -> Scope/1
  Gain5/1 -> Scope/2
  [Igrid] -> Gain5/1
  NOT3/1 -> Scope7/4
  NOT2/1 -> Scope7/2
  [Vout] -> Scope/3
  [Q1H] -> NOT2/1, Scope7/1
  [PF] -> Scope8/1
  [Q2H] -> NOT3/1, Scope7/3
  [Igrid] -> Scope5/2
  [Vo] -> Scope5/4
  [coswt] -> Scope2/4
  [Iinv] -> Scope5/1
  [PWM4] -> Scope4/4
  [ON] -> Scope6/2
  [Sync] -> Scope6/1
  [PWM1] -> Scope4/1
  [sinwt] -> Scope2/5
  [Vinv] -> Scope5/3
  [Vq] -> Scope2/2
  [Iref] -> Scope3/1
  [PWM2] -> Scope4/2
  [Igrid] -> Scope3/2
  [Vgrid] -> Scope2/1
  [Wt] -> Scope2/3
  [PWM3] -> Scope4/3
  Switch9/1 -> [Q1H]
  Abs1/1 -> Multiply1/2
  PID Controller1/1 -> Multiply1/1
  Gain11/1 -> [PWM22]
  [Vout] -> Sum6/2
  Constant1/1 -> Switch10/3
  Gain4/1 -> Switch5/1
  Sum7/1 -> PID Controller4/1
  Constant5/1 -> Switch10/1
  Multiply1/1 -> Sum7/1
  Constant2/1 -> GreaterThanOrEqual5/2
  Sum6/1 -> PID Controller1/1
  GreaterThanOrEqual5/1 -> Switch10/2, Switch9/2, [H]
  [PWM11] -> Switch9/3
  [Vgrid] -> GreaterThanOrEqual5/1
  [I] -> Sum7/2
  Switch5/1 -> [I]
  [Igrid] -> Gain4/1
  [Igrid] -> Switch5/3
  [H] -> Switch5/2
  Saturation3/1 -> Sum6/1
  [Vgrid] -> Gain3/1
  Switch10/1 -> Scope20/1, [Q2H]
  [PWM22] -> Switch9/1
  Ramp1/1 -> Saturation3/1
  PID Controller4/1 -> Gain11/1, [PWM11]
  Gain3/1 -> Abs1/1
  Gain12/1 -> Product2/2, Product4/2, Product4/1
  Product1/1 -> Add1/1
  Add1/1 -> Divide3/2
  Sqrt1/1 -> Product1/2
  Transfer Fcn/1 -> Divide3/1
  [Igrid] -> Gain12/1
  Product3/1 -> Transfer Fcn1/1
  Product2/1 -> Transfer Fcn/1
  Transfer Fcn1/1 -> Sqrt/1
  Transfer Fcn2/1 -> Sqrt1/1
  [Vgrid] -> Product2/1, Product3/2, Product3/1
  Divide3/1 -> [PF]
  Product4/1 -> Transfer Fcn2/1
  Constant20/1 -> Add1/2
  Sqrt/1 -> Product1/1
  Gain6/1 -> Sum9/1  "-Vref"
  Constant17/1 -> Sum9/2
  [ON] -> Switch1/2
  Gain1/1 -> Switch1/3
  Constant16/1 -> Sum8/2
  [Vref] -> Switch1/1
  [coswt] -> Gain1/1
  Sum8/1 -> Gain17/1
  Gain18/1 -> [PWM3]
  Sum9/1 -> Gain18/1
  Switch1/1 -> Sum8/1, Gain6/1
  Gain17/1 -> [PWM1]
  [ePWM4B] -> Scope1/4
  [ePWM4A] -> Scope1/3
  [ePWM2B] -> Scope1/2
  [ePWM2A] -> Scope1/1
  Logical Operator3/1 -> Logical Operator2/1
  [Sync] -> Logical Operator2/2
  Switch8/1 -> [Ts]
  [X] -> Switch8/2
  f100kHz/1 -> Switch8/1
  f10kHztant2/1 -> Switch8/3
